simulink model "simulink_start"  (R2026a)
settings: Solver=VariableStepAuto  StopTime=5
undefined symbols (not defined in the file): k, m
settings Model: Creator=zsoltikv  LastModifiedBy=zsoltikv

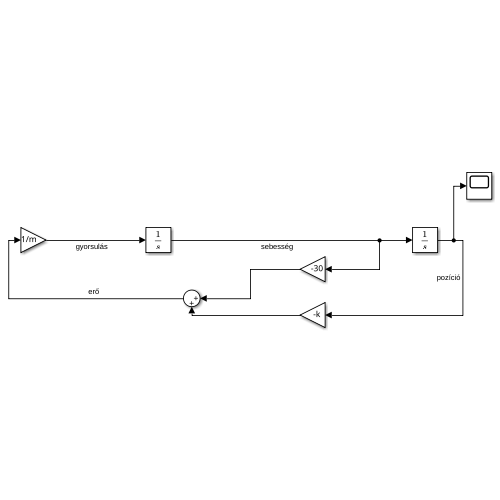
[thumbnail: Simulink's stored preview of the top-level diagram]
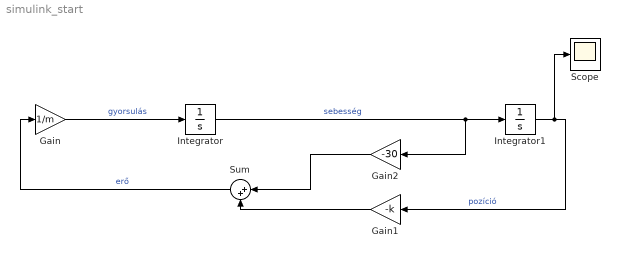
== system simulink_start ==
  Gain : Gain  Gain=1/m
  Gain1 : Gain  Gain=-k
  Gain2 : Gain  Gain=-30
  Integrator : Integrator
  Integrator1 : Integrator  InitialCondition=1
  Scope : Scope
      settings: ActiveDisplayYMinimum=-0.49245272776330817  ActiveDisplayYMaximum=1.1658280808625898
  Sum : Sum  Inputs=|++
  wires:
  Gain/1 -> Integrator/1  "gyorsulás"
  Integrator/1 -> Gain2/1, Integrator1/1  "sebesség"
  Integrator1/1 -> Scope/1, Gain1/1  "pozíció"
  Gain2/1 -> Sum/1
  Gain1/1 -> Sum/2
  Sum/1 -> Gain/1  "erő"
